simulink model "Tractor_HIT_Discrete"  (R2024a)
settings: Solver=ode1  StartTime=0.0  StopTime=60  FixedStep=0.001  RelTol=1e-3
values from neighbouring files (symbols this model uses):
  ANRtarget = 1.05    [Engine1204.sldd]    (also in Engine1204_init_r1.m; Engine2004.sldd; Engine2004_init.m; Engine3204.sldd)
  BackPrs = 3.0 4.2 5.5 7.0 8.5 10.0 11.5 12.5    [Engine1204.sldd]    (also in Engine1204_init_r1.m = [3.0, 4.2, 5.5, 7.0, 8.5, 10.0, 11.5, 12.5]; Engine2004.sldd = 3.0 4.2 5.5 7.0 8.5 10.0 11.5 12.5 13.5 14.5 15.0 15.5 16.0 ; Engine2004_init.m = [3.0,4.2,5.5,7.0,8.5,10.0,11.5,12.5,13.5,14.5,15.0,15.5,16.0; Engine3204.sldd = 3.0 4.5 6.0 7.5 9.0 10.5 12.0 13.0 13.8 14.4 14.8 15.2 15.6 )
  BackPrs_x = 50.0 100.0 150.0 200.0 250.0 300.0 350.0 400.0    [Engine1204.sldd]    (also in Engine1204_init_r1.m = [50:50:400]; Engine2004.sldd = 50.0 100.0 150.0 200.0 250.0 300.0 350.0 400.0 450.0 500.0 5; Engine2004_init.m = [50:50:800]; Engine3204.sldd = 100.0 200.0 300.0 400.0 500.0 600.0 700.0 800.0 900.0 1000.0)
  Bf = 0.38    [Engine1204.sldd]    (also in Engine2004.sldd; Engine3204.sldd)
  Br = 0.47    [Engine1204.sldd]    (also in Engine2004.sldd; Engine3204.sldd)
  BSFC = 320.0 285.0 275.0 280.0 290.0 300.0 310.0 260.0 225.0 215.0 220.0 228.0 240.0 250.0 235.0 208.0 202.0 205.0 212.0 222.0 232.0 230.0 205.0 200.0 204.0 210.0 220.0 230.0 232.0 207.0 203.0 206.0 213.0 224.0 235.0    [Engine1204.sldd]    (also in Engine1204_init_r1.m = [320,285,275,280,290,300,310; Engine2004.sldd = 315.0 280.0 270.0 275.0 285.0 295.0 305.0 255.0 220.0 210.0 ; Engine2004_init.m = [315,280,270,275,285,295,305; Engine3204.sldd = 310.0 275.0 265.0 270.0 280.0 290.0 300.0 250.0 215.0 205.0 )
  BSFC_x = 700.0 1200.0 1400.0 1600.0 1800.0 2000.0 2200.0    [Engine1204.sldd]    (also in Engine1204_init_r1.m = [700,1200,1400,1600,1800,2000,2200]; Engine2004.sldd = 800.0 1200.0 1400.0 1600.0 1800.0 2000.0 2200.0; Engine2004_init.m = [800,1200,1400,1600,1800,2000,2200]; Engine3204.sldd = 800.0 1000.0 1200.0 1400.0 1600.0 1800.0 2100.0)
  BSFC_y = 12.0 24.0 36.0 48.0 54.0    [Engine1204.sldd]    (also in Engine1204_init_r1.m = [12,24,36,48,54]; Engine2004.sldd = 20.0 40.0 60.0 80.0 100.0; Engine2004_init.m = [20,40,60,80,100]; Engine3204.sldd = 30.0 60.0 90.0 120.0 150.0)
  CO = 2.4 1.7 1.5 1.6 1.8 2.1 2.7 1.1 0.72 0.65 0.68 0.78 0.92 1.3 0.7 0.55 0.5 0.53 0.6 0.72 0.95 1.2 0.9 0.85 0.88 0.96 1.1 1.45 3.2 2.3 2.1 2.25 2.5 2.85 3.8    [Engine1204.sldd]    (also in Engine1204_init_r1.m = [; Engine2004.sldd = 2.3 1.63 1.44 1.54 1.73 2.02 2.56 1.05 0.68 0.61 0.64 0.74 0; Engine2004_init.m = [; Engine3204.sldd = 2.2 1.56 1.38 1.48 1.66 1.94 2.46 1.0 0.65 0.58 0.61 0.7 0.8)
  CO_x = 700.0 1200.0 1400.0 1600.0 1800.0 2000.0 2200.0    [Engine1204.sldd]    (also in Engine1204_init_r1.m = [700,1200,1400,1600,1800,2000,2200]; Engine2004.sldd = 800.0 1200.0 1400.0 1600.0 1800.0 2000.0 2200.0; Engine2004_init.m = [800,1200,1400,1600,1800,2000,2200]; Engine3204.sldd = 800.0 1000.0 1200.0 1400.0 1600.0 1800.0 2100.0)
  CO_y = 12.0 24.0 36.0 48.0 54.0    [Engine1204.sldd]    (also in Engine1204_init_r1.m = [12,24,36,48,54]; Engine2004.sldd = 20.0 40.0 60.0 80.0 100.0; Engine2004_init.m = [20,40,60,80,100]; Engine3204.sldd = 30.0 60.0 90.0 120.0 150.0)
  Df = 1.4    [Engine1204.sldd]    (also in Engine2004.sldd; Engine3204.sldd)
  dfmax = 0.1    [Engine1204.sldd]    (also in Engine2004.sldd; Engine3204.sldd)
  dfmin = 0.035    [Engine1204.sldd]    (also in Engine2004.sldd; Engine3204.sldd)
  DOCdPrs = 0.2 0.5 0.8 1.1 1.2    [Engine1204.sldd]    (also in Engine1204_init_r1.m = [0.2  0.5  0.8  1.1  1.2]; Engine2004.sldd = 0.25 0.55 0.85 1.15 1.3; Engine2004_init.m = [0.25,0.55,0.85,1.15,1.30]; Engine3204.sldd = 0.25 0.55 0.85 1.15 1.3 1.45)
  DOCdPrs_x = 50.0 150.0 250.0 350.0 400.0    [Engine1204.sldd]    (also in Engine1204_init_r1.m = [50  150  250  350  400]; Engine2004.sldd = 100.0 250.0 400.0 600.0 800.0; Engine2004_init.m = [100 250 400 600 800]; Engine3204.sldd = 100.0 250.0 400.0 600.0 800.0 1200.0)
  DPFdPrs = 0.3 0.5 0.7 0.9 0.6 1.0 1.4 1.8 0.9 1.5 2.1 2.6 1.2 2.0 2.7 2.8    [Engine1204.sldd]    (also in Engine1204_init_r1.m = [0.3  0.5  0.7  0.9; Engine2004.sldd = 0.35 0.6 0.85 1.1 0.7 1.15 1.6 2.0 1.05 1.7 2.3 2.5 1.4 2.2 ; Engine2004_init.m = [0.35,0.60,0.85,1.10; Engine3204.sldd = 0.35 0.7 1.05 1.4 1.7 2.0 2.2 2.4 2.55 2.65 2.7 2.75 0.6 1.1)
  DPFdPrs_x = 100.0 200.0 300.0 400.0    [Engine1204.sldd]    (also in Engine1204_init_r1.m = [100: 100 : 400]; Engine2004.sldd = 100.0 300.0 500.0 700.0; Engine2004_init.m = [100:200:700]; Engine3204.sldd = 100.0 200.0 300.0 400.0 500.0 600.0 700.0 800.0 900.0 1000.0)
  DPFdPrs_y = 0.0 6.0 12.0 20.0    [Engine1204.sldd]    (also in Engine1204_init_r1.m = [0 6 12 20 ]; Engine2004.sldd = 0.0 8.0 16.0 24.0; Engine2004_init.m = [0 8 16 24]; Engine3204.sldd = 0.0 10.0 20.0 30.0)
  DPFSootBurn = 0.0 0.0 0.0 0.0 0.0 0.2 0.4 0.6 0.8 1.0 1.2 2.4 3.6 4.8 6.0 6.0 12.0 18.0 24.0 30.0 12.0 24.0 36.0 48.0 60.0 20.0 40.0 60.0 80.0 100.0 22.0 44.0 66.0 88.0 110.0    [Engine1204.sldd]    (also in Engine1204_init_r1.m = [0,0,0,0,0; Engine2004.sldd = 0.0 0.0 0.0 0.0 0.0 0.5 1.0 1.5 2.0 2.5 3.0 6.0 9.0 12.0 15.; Engine2004_init.m = [0,0,0,0,0; Engine3204.sldd = 0.0 0.0 0.0 0.0 0.0 0.5 1.0 1.5 2.0 2.5 3.0 6.0 9.0 12.0 15.)
  DPFSootBurn_x = 100.0 200.0 300.0 400.0 500.0    [Engine1204.sldd]    (also in Engine1204_init_r1.m = [100,200,300,400,500]; Engine2004.sldd = 200.0 300.0 400.0 500.0 650.0; Engine2004_init.m = [200,300,400,500,650]; Engine3204.sldd = 200.0 300.0 400.0 500.0 650.0)
  DPFSootBurn_y = 400.0 450.0 500.0 550.0 600.0 650.0 680.0    [Engine1204.sldd]    (also in Engine1204_init_r1.m = [400,450,500,550,600,650,680]; Engine2004.sldd; Engine2004_init.m = [400,450,500,550,600,650,680]; Engine3204.sldd)
  Dr = 1.8    [Engine1204.sldd]    (also in Engine2004.sldd; Engine3204.sldd)
  drmax = 0.12    [Engine1204.sldd]    (also in Engine2004.sldd; Engine3204.sldd)
  drmin = 0.04    [Engine1204.sldd]    (also in Engine2004.sldd; Engine3204.sldd)
  EGRKi = 0.03    [Engine1204.sldd]    (also in Engine1204_init_r1.m; Engine2004.sldd; Engine2004_init.m; Engine3204.sldd)
  EGRKp = 3.5999999999999996    [Engine1204.sldd]    (also in Engine1204_init_r1.m = 3.6; Engine2004.sldd; Engine2004_init.m = 3.6; Engine3204.sldd)
  EGRMax = 1.0    [Engine1204.sldd]    (also in Engine1204_init_r1.m = 1; Engine2004.sldd; Engine2004_init.m = 1; Engine3204.sldd)
  EGRMin = 0.0    [Engine1204.sldd]    (also in Engine1204_init_r1.m = 0; Engine2004.sldd; Engine2004_init.m = 0; Engine3204.sldd)
  EGRRatio = 0.0 0.0 0.0 0.0 0.0 0.0 0.0 0.0 0.04 0.03 0.03 0.02 0.02 0.01 0.0 0.08 0.07 0.06 0.05 0.04 0.03 0.0 0.13 0.12 0.11 0.1 0.09 0.08 0.0 0.18 0.17 0.16 0.15 0.14 0.13 0.0 0.22 0.21 0.2 0.19 0.18 0.17    [Engine1204.sldd]    (also in Engine1204_init_r1.m = [; Engine2004.sldd; Engine2004_init.m = [; Engine3204.sldd)
  EGRRatio_x = 700.0 1200.0 1400.0 1600.0 1800.0 2000.0 2200.0    [Engine1204.sldd]    (also in Engine1204_init_r1.m = [700,1200,1400,1600,1800,2000,2200]; Engine2004.sldd = 800.0 1200.0 1400.0 1600.0 1800.0 2000.0 2200.0; Engine2004_init.m = [800,1200,1400,1600,1800,2000,2200]; Engine3204.sldd = 800.0 1000.0 1200.0 1400.0 1600.0 1800.0 2100.0)
  EGRRatio_y = 0.0 20.0 40.0 60.0 80.0 100.0    [Engine1204.sldd]    (also in Engine1204_init_r1.m = [0,20,40,60,80,100]; Engine2004.sldd; Engine2004_init.m = [0,20,40,60,80,100]; Engine3204.sldd)
  EGRTgt = 0.25 0.22 0.2 0.18 0.16 0.12 0.1 0.2 0.18 0.15 0.14 0.12 0.1 0.08 0.12 0.13 0.1 0.09 0.08 0.06 0.04 0.08 0.09 0.07 0.06 0.05 0.03 0.02 0.05 0.06 0.04 0.03 0.02 0.01 0.0    [Engine1204.sldd]    (also in Engine1204_init_r1.m = [0.25,0.22,0.20,0.18,0.16,0.12,0.10; Engine2004.sldd = 0.24 0.21 0.19 0.17 0.15 0.11 0.09 0.19 0.17 0.14 0.13 0.11 ; Engine2004_init.m = [0.24,0.21,0.19,0.17,0.15,0.11,0.09; Engine3204.sldd = 0.23 0.2 0.18 0.16 0.14 0.1 0.08 0.18 0.16 0.13 0.12 0.1 0.0)
  EGRTgt_x = 700.0 1200.0 1400.0 1600.0 1800.0 2000.0 2200.0    [Engine1204.sldd]    (also in Engine1204_init_r1.m = [700,1200,1400,1600,1800,2000,2200]; Engine2004.sldd = 800.0 1200.0 1400.0 1600.0 1800.0 2000.0 2200.0; Engine2004_init.m = [800,1200,1400,1600,1800,2000,2200]; Engine3204.sldd = 800.0 1000.0 1200.0 1400.0 1600.0 1800.0 2100.0)
  EGRTgt_y = 12.0 24.0 36.0 48.0 54.0    [Engine1204.sldd]    (also in Engine1204_init_r1.m = [12,24,36,48,54]; Engine2004.sldd = 20.0 40.0 60.0 80.0 100.0; Engine2004_init.m = [20,40,60,80,100]; Engine3204.sldd = 30.0 60.0 90.0 120.0 150.0)
  EGT = 197.0 257.0 287.0 297.0 287.0 267.0 247.0 267.0 357.0 397.0 407.0 392.0 367.0 347.0 337.0 437.0 472.0 482.0 462.0 437.0 407.0 367.0 477.0 502.0 512.0 492.0 467.0 437.0 377.0 487.0 510.0 520.0 500.0 477.0 447.0    [Engine1204.sldd]    (also in Engine1204_init_r1.m = [470,530,560,570,560,540,520; Engine2004.sldd = 187.0 247.0 277.0 287.0 277.0 257.0 237.0 257.0 347.0 387.0 ; Engine2004_init.m = [460,520,550,560,550,530,510; Engine3204.sldd = 307.0 327.0 338.0 327.0 307.0 277.0 237.0 322.0 337.0 332.0 )
  EGT_x = 700.0 1200.0 1400.0 1600.0 1800.0 2000.0 2200.0    [Engine1204.sldd]    (also in Engine1204_init_r1.m = [700,1200,1400,1600,1800,2000,2200]; Engine2004.sldd = 800.0 1200.0 1400.0 1600.0 1800.0 2000.0 2200.0; Engine2004_init.m = [800,1200,1400,1600,1800,2000,2200]; Engine3204.sldd = 800.0 1000.0 1200.0 1400.0 1600.0 1800.0 2100.0)
  EGT_y = 12.0 24.0 36.0 48.0 54.0    [Engine1204.sldd]    (also in Engine1204_init_r1.m = [12,24,36,48,54]; Engine2004.sldd = 20.0 40.0 60.0 80.0 100.0; Engine2004_init.m = [20,40,60,80,100]; Engine3204.sldd = 30.0 60.0 90.0 120.0 150.0)
  EngCsup = 0.35594 0.35501499999999997 0.353535 0.35242500000000004 0.351685 0.35150000000000003 0.35187 0.352795 0.35446 0.356865    [Engine1204.sldd]    (also in Engine2004.sldd; Engine3204.sldd)
  EngineSpdTgt = 700.0 850.0 1000.0 1150.0 1300.0 1450.0 1600.0 1750.0 1900.0 2050.0 2200.0    [Engine1204.sldd]    (also in Engine1204_init_r1.m = [700:150:2200]; Engine2004.sldd; Engine2004_init.m = [700:150:2200]; Engine3204.sldd = 800.0 930.0 1060.0 1190.0 1320.0 1450.0 1580.0 1710.0 1840.0)
  EngineSpdTgt_x = 0.0 10.0 20.0 30.0 40.0 50.0 60.0 70.0 80.0 90.0 100.0    [Engine1204.sldd]    (also in Engine1204_init_r1.m = [0:10:100]; Engine2004.sldd; Engine2004_init.m = [0:10:100]; Engine3204.sldd)
  EngineTrq = 70.0 110.0 130.0 125.0 115.0 100.0 85.0 180.0 280.0 320.0 310.0 285.0 250.0 220.0 260.0 370.0 410.0 395.0 365.0 320.0 280.0 300.0 420.0 450.0 435.0 400.0 350.0 300.0 310.0 435.0 460.0 445.0 410.0 355.0 305.0    [Engine1204.sldd]    (also in Engine1204_init_r1.m = [70,110,130,125,115,100,85; Engine2004.sldd = 130.0 200.0 240.0 230.0 210.0 180.0 150.0 320.0 480.0 550.0 ; Engine2004_init.m = [130,200,240,230,210,180,150; Engine3204.sldd = 210.0 320.0 380.0 360.0 330.0 290.0 240.0 510.0 760.0 870.0 )
  EngineTrq_x = 700.0 1200.0 1400.0 1600.0 1800.0 2000.0 2200.0    [Engine1204.sldd]    (also in Engine1204_init_r1.m = [700,1200,1400,1600,1800,2000,2200]; Engine2004.sldd = 800.0 1200.0 1400.0 1600.0 1800.0 2000.0 2200.0; Engine2004_init.m = [800,1200,1400,1600,1800,2000,2200]; Engine3204.sldd = 800.0 1000.0 1200.0 1400.0 1600.0 1800.0 2100.0)
  EngineTrq_y = 12.0 24.0 36.0 48.0 54.0    [Engine1204.sldd]    (also in Engine1204_init_r1.m = [12,24,36,48,54]; Engine2004.sldd = 20.0 40.0 60.0 80.0 100.0; Engine2004_init.m = [20,40,60,80,100]; Engine3204.sldd = 30.0 60.0 90.0 120.0 150.0)
  EngSpd = 800.0 1000.0 1200.0 1400.0 1600.0 1800.0 2000.0 2200.0 2400.0 2600.0    [Engine1204.sldd]    (also in Engine2004.sldd; Engine3204.sldd)
  EngTrq = 667.0 700.0 768.0 830.0 885.0 860.0 789.0 690.0 542.0 352.0    [Engine1204.sldd]    (also in Engine2004.sldd; Engine3204.sldd)
  etaCO = 0.0 0.0 0.0 0.0 0.6 0.45 0.3 0.15 0.92 0.85 0.75 0.6 0.98 0.95 0.9 0.82 0.99 0.97 0.94 0.88    [Engine1204.sldd]    (also in Engine1204_init_r1.m = [0.00	0.00	0.00	0.00; Engine2004.sldd; Engine2004_init.m = [0.00	0.00	0.00	0.00; Engine3204.sldd)
  etaCO_x = 10000.0 25000.0 40000.0 60000.0    [Engine1204.sldd]    (also in Engine1204_init_r1.m = [10000  25000  40000  60000]; Engine2004.sldd; Engine2004_init.m = [10000 25000 40000 60000]; Engine3204.sldd)
  etaCO_y = 120.0 200.0 280.0 360.0 450.0    [Engine1204.sldd]    (also in Engine1204_init_r1.m = [120, 200, 280, 360, 450]; Engine2004.sldd; Engine2004_init.m = [120,200,280,360,450]; Engine3204.sldd)
  etaHC = 0.0 0.0 0.0 0.0 0.5 0.35 0.2 0.1 0.88 0.8 0.68 0.5 0.96 0.92 0.86 0.75 0.98 0.95 0.91 0.83    [Engine1204.sldd]    (also in Engine1204_init_r1.m = [0.00	0.00	0.00	0.00; Engine2004.sldd; Engine2004_init.m = [0.00	0.00	0.00	0.00; Engine3204.sldd)
  etaHC_x = 10000.0 25000.0 40000.0 60000.0    [Engine1204.sldd]    (also in Engine1204_init_r1.m = [10000  25000  40000  60000]; Engine2004.sldd; Engine2004_init.m = [10000 25000 40000 60000]; Engine3204.sldd)
  etaHC_y = 120.0 200.0 280.0 360.0 450.0    [Engine1204.sldd]    (also in Engine1204_init_r1.m = [120, 200, 280, 360, 450]; Engine2004.sldd; Engine2004_init.m = [120,200,280,360,450]; Engine3204.sldd)
  etaNO2 = 0.0 0.0 0.0 0.0 0.2 0.15 0.1 0.05 0.4 0.33 0.25 0.18 0.55 0.48 0.4 0.3 0.6 0.53 0.45 0.35    [Engine1204.sldd]    (also in Engine1204_init_r1.m = [0.00	0.00	0.00	0.00; Engine2004.sldd; Engine2004_init.m = [0.00	0.00	0.00	0.00; Engine3204.sldd)
  etaNO2_x = 10000.0 25000.0 40000.0 60000.0    [Engine1204.sldd]    (also in Engine1204_init_r1.m = [10000  25000  40000  60000]; Engine2004.sldd; Engine2004_init.m = [10000 25000 40000 60000]; Engine3204.sldd)
  etaNO2_y = 120.0 200.0 280.0 360.0 450.0    [Engine1204.sldd]    (also in Engine1204_init_r1.m = [120, 200, 280, 360, 450]; Engine2004.sldd; Engine2004_init.m = [120,200,280,360,450]; Engine3204.sldd)
  etaPM = 0.995 0.992 0.988 0.98 0.996 0.994 0.99 0.985 0.997 0.995 0.992 0.988    [Engine1204.sldd]    (also in Engine1204_init_r1.m = [0.995  0.992  0.988  0.980; Engine2004.sldd; Engine2004_init.m = [0.995  0.992  0.988  0.980; Engine3204.sldd)
  etaPM_x = 10000.0 25000.0 40000.0 60000.0    [Engine1204.sldd]    (also in Engine1204_init_r1.m = [10000  25000  40000  60000]; Engine2004.sldd; Engine2004_init.m = [10000 25000 40000 60000]; Engine3204.sldd)
  etaPM_y = 150.0 300.0 450.0    [Engine1204.sldd]    (also in Engine1204_init_r1.m = [150, 300, 450]; Engine2004.sldd; Engine2004_init.m = [150,300,450]; Engine3204.sldd)
  FuelCyleMax = 40.0 45.0 50.0 52.0 54.0 50.0 60.0 65.0 66.0 68.0 52.0 64.0 66.0 67.0 68.0 50.0 62.0 64.0 65.0 66.0 48.0 58.0 60.0 61.0 62.0 42.0 50.0 52.0 53.0 54.0 38.0 44.0 46.0 47.0 48.0    [Engine1204.sldd]    (also in Engine1204_init_r1.m = [40,45,50,52,54; Engine2004.sldd = 65.0 75.0 82.0 88.0 92.0 75.0 88.0 94.0 98.0 102.0 78.0 92.0; Engine2004_init.m = [65,75,82,88,92; Engine3204.sldd = 95.0 110.0 125.0 140.0 155.0 110.0 130.0 145.0 160.0 175.0 1)
  FuelCyleMax_x = 80.0 140.0 200.0 260.0 320.0    [Engine1204.sldd]    (also in Engine1204_init_r1.m = [80,140,200,260,320]; Engine2004.sldd = 150.0 300.0 450.0 600.0 750.0; Engine2004_init.m = [150,300,450,600,750]; Engine3204.sldd = 250.0 500.0 750.0 1000.0 1300.0)
  FuelCyleMax_y = 700.0 1200.0 1400.0 1600.0 1800.0 2000.0 2200.0    [Engine1204.sldd]    (also in Engine1204_init_r1.m = [700,1200,1400,1600,1800,2000,2200]; Engine2004.sldd = 800.0 1200.0 1400.0 1600.0 1800.0 2000.0 2200.0; Engine2004_init.m = [800,1200,1400,1600,1800,2000,2200]; Engine3204.sldd = 800.0 1000.0 1200.0 1400.0 1600.0 1800.0 2100.0)
  FuelCyleMaxSw = 0.0    [Engine1204.sldd]    (also in Engine1204_init_r1.m = 0; Engine2004.sldd; Engine2004_init.m = 0; Engine3204.sldd)
  FuelCyleMin = 10.0    [Engine1204.sldd]    (also in Engine1204_init_r1.m = 10; Engine2004.sldd = 12.0; Engine2004_init.m = 12; Engine3204.sldd = 15.0)
  FuelKd = 0.0    [Engine1204.sldd]    (also in Engine1204_init_r1.m = 0; Engine2004.sldd; Engine2004_init.m = 0; Engine3204.sldd)
  FuelKi = 0.0162    [Engine1204.sldd]    (also in Engine1204_init_r1.m; Engine2004.sldd = 0.0198; Engine2004_init.m = 0.0198; Engine3204.sldd = 0.025199999999999997)
  FuelKp = 0.054    [Engine1204.sldd]    (also in Engine1204_init_r1.m; Engine2004.sldd = 0.066; Engine2004_init.m = 0.066; Engine3204.sldd = 0.083999999999999991)
  g = 9.81    [Engine1204.sldd]    (also in Engine2004.sldd; Engine3204.sldd)
  GearA = -2.9 0.0 6.0 2.5 1.0    [Engine1204.sldd]    (also in Engine2004.sldd; Engine3204.sldd)
  GearAC = -1.0 0.0 1.0 2.0 3.0    [Engine1204.sldd]    (also in Engine2004.sldd; Engine3204.sldd)
  GearFront = 17.574    [Engine1204.sldd]    (also in Engine2004.sldd; Engine3204.sldd)
  GearM = 2.33 1.75 1.4 1.0    [Engine1204.sldd]    (also in Engine2004.sldd; Engine3204.sldd)
  GearMC = 1.0 2.0 3.0 4.0    [Engine1204.sldd]    (also in Engine2004.sldd; Engine3204.sldd)
  GearRef = 14.6    [Engine1204.sldd]    (also in Engine2004.sldd; Engine3204.sldd)
  HC = 0.85 0.6 0.52 0.55 0.62 0.7 0.9 0.4 0.22 0.2 0.21 0.26 0.32 0.48 0.25 0.18 0.17 0.18 0.21 0.26 0.36 0.32 0.24 0.23 0.25 0.28 0.33 0.42 0.55 0.42 0.4 0.43 0.48 0.54 0.68    [Engine1204.sldd]    (also in Engine1204_init_r1.m = [; Engine2004.sldd = 0.82 0.58 0.5 0.53 0.6 0.68 0.87 0.38 0.21 0.19 0.2 0.24 0.3; Engine2004_init.m = [; Engine3204.sldd = 0.8 0.56 0.48 0.51 0.58 0.66 0.84 0.37 0.2 0.18 0.19 0.23 0.)
  HC_x = 700.0 1200.0 1400.0 1600.0 1800.0 2000.0 2200.0    [Engine1204.sldd]    (also in Engine1204_init_r1.m = [700,1200,1400,1600,1800,2000,2200]; Engine2004.sldd = 800.0 1200.0 1400.0 1600.0 1800.0 2000.0 2200.0; Engine2004_init.m = [800,1200,1400,1600,1800,2000,2200]; Engine3204.sldd = 800.0 1000.0 1200.0 1400.0 1600.0 1800.0 2100.0)
  HC_y = 12.0 24.0 36.0 48.0 54.0    [Engine1204.sldd]    (also in Engine1204_init_r1.m = [12,24,36,48,54]; Engine2004.sldd = 20.0 40.0 60.0 80.0 100.0; Engine2004_init.m = [20,40,60,80,100]; Engine3204.sldd = 30.0 60.0 90.0 120.0 150.0)
  hf = 0.35    [Engine1204.sldd]    (also in Engine2004.sldd; Engine3204.sldd)
  hr = 0.4    [Engine1204.sldd]    (also in Engine2004.sldd; Engine3204.sldd)
  IdleEngSpd = 700.0    [Engine1204.sldd]    (also in Engine2004.sldd; Engine3204.sldd)
  IdleThrottle = 0.3    [Engine1204.sldd]    (also in Engine2004.sldd; Engine3204.sldd)
  Inertia = 0.9    [Engine1204.sldd]    (also in Engine1204_init_r1.m; Engine2004.sldd = 1.4; Engine2004_init.m = 1.4; Engine3204.sldd = 2.0)
  Intake = 80.0 140.0 160.0 180.0 190.0 195.0 200.0 130.0 210.0 240.0 260.0 270.0 275.0 280.0 170.0 270.0 310.0 330.0 340.0 345.0 350.0 190.0 320.0 360.0 380.0 390.0 395.0 400.0 200.0 340.0 380.0 400.0 410.0 415.0 420.0    [Engine1204.sldd]    (also in Engine1204_init_r1.m = [80,140,160,180,190,195,200; Engine2004.sldd = 160.0 240.0 280.0 310.0 330.0 340.0 350.0 250.0 380.0 440.0 ; Engine2004_init.m = [160,240,280,310,330,340,350; Engine3204.sldd = 280.0 420.0 490.0 540.0 570.0 585.0 600.0 430.0 660.0 760.0 )
  Intake_x = 700.0 1200.0 1400.0 1600.0 1800.0 2000.0 2200.0    [Engine1204.sldd]    (also in Engine1204_init_r1.m = [700,1200,1400,1600,1800,2000,2200]; Engine2004.sldd = 800.0 1200.0 1400.0 1600.0 1800.0 2000.0 2200.0; Engine2004_init.m = [800,1200,1400,1600,1800,2000,2200]; Engine3204.sldd = 800.0 1000.0 1200.0 1400.0 1600.0 1800.0 2100.0)
  Intake_y = 12.0 24.0 36.0 48.0 54.0    [Engine1204.sldd]    (also in Engine1204_init_r1.m = [12,24,36,48,54]; Engine2004.sldd = 20.0 40.0 60.0 80.0 100.0; Engine2004_init.m = [20,40,60,80,100]; Engine3204.sldd = 30.0 60.0 90.0 120.0 150.0)
  IntakePrs = 1.0 1.1 1.22 1.35 1.48 1.6 1.7 1.0 1.12 1.24 1.37 1.5 1.62 1.72 1.0 1.13 1.25 1.38 1.51 1.63 1.73 1.0 1.14 1.26 1.39 1.52 1.64 1.74 1.0 1.15 1.27 1.4 1.53 1.65 1.75 1.0 1.16 1.28 1.41 1.54 1.66 1.76    [Engine1204.sldd]    (also in Engine1204_init_r1.m = [; Engine2004.sldd = 1.0 1.11 1.23 1.36 1.49 1.61 1.71 1.0 1.13 1.25 1.38 1.51 1.; Engine2004_init.m = [; Engine3204.sldd = 1.0 1.12 1.24 1.37 1.5 1.62 1.72 1.0 1.14 1.26 1.39 1.52 1.6)
  IntakePrs_x = 700.0 1200.0 1400.0 1600.0 1800.0 2000.0 2200.0    [Engine1204.sldd]    (also in Engine1204_init_r1.m = [700,1200,1400,1600,1800,2000,2200]; Engine2004.sldd = 800.0 1200.0 1400.0 1600.0 1800.0 2000.0 2200.0; Engine2004_init.m = [800,1200,1400,1600,1800,2000,2200]; Engine3204.sldd = 800.0 1000.0 1200.0 1400.0 1600.0 1800.0 2100.0)
  IntakePrs_y = 0.0 20.0 40.0 60.0 80.0 100.0    [Engine1204.sldd]    (also in Engine1204_init_r1.m = [0,20,40,60,80,100]; Engine2004.sldd; Engine2004_init.m = [0,20,40,60,80,100]; Engine3204.sldd)
  IntakePrsInit = 1.35    [Engine1204.sldd]    (also in Engine1204_init_r1.m; Engine2004.sldd; Engine2004_init.m; Engine3204.sldd)
  IntakeSw = 0    [Engine1204.sldd]    (also in Engine1204_init_r1.m = false; Engine2004.sldd; Engine2004_init.m = false; Engine3204.sldd)
  IntakeTC = 0.1    [Engine1204.sldd]    (also in Engine1204_init_r1.m; Engine2004.sldd; Engine2004_init.m; Engine3204.sldd)
  IntakeTemp = 25.0 28.0 30.0 32.0 34.0 36.0 38.0 25.0 38.0 40.0 42.0 44.0 46.0 48.0 25.0 48.0 50.0 52.0 54.0 56.0 58.0 25.0 58.0 60.0 62.0 64.0 66.0 68.0 25.0 66.0 68.0 70.0 72.0 74.0 76.0 25.0 72.0 74.0 76.0 78.0 80.0 82.0    [Engine1204.sldd]    (also in Engine1204_init_r1.m = [; Engine2004.sldd = 25.0 29.0 31.0 33.0 35.0 37.0 39.0 25.0 39.0 41.0 43.0 45.0 ; Engine2004_init.m = [; Engine3204.sldd = 25.0 30.0 32.0 34.0 36.0 38.0 40.0 25.0 40.0 42.0 44.0 46.0 )
  IntakeTemp_x = 700.0 1200.0 1400.0 1600.0 1800.0 2000.0 2200.0    [Engine1204.sldd]    (also in Engine1204_init_r1.m = [700,1200,1400,1600,1800,2000,2200]; Engine2004.sldd = 800.0 1200.0 1400.0 1600.0 1800.0 2000.0 2200.0; Engine2004_init.m = [800,1200,1400,1600,1800,2000,2200]; Engine3204.sldd = 800.0 1000.0 1200.0 1400.0 1600.0 1800.0 2100.0)
  IntakeTemp_y = 0.0 20.0 40.0 60.0 80.0 100.0    [Engine1204.sldd]    (also in Engine1204_init_r1.m = [0,20,40,60,80,100]; Engine2004.sldd; Engine2004_init.m = [0,20,40,60,80,100]; Engine3204.sldd)
  IntakeTempInit = 45.0    [Engine1204.sldd]    (also in Engine1204_init_r1.m = 45; Engine2004.sldd; Engine2004_init.m = 45; Engine3204.sldd)
  Jf = 180.0    [Engine1204.sldd]    (also in Engine2004.sldd; Engine3204.sldd)
  Jr = 450.0    [Engine1204.sldd]    (also in Engine2004.sldd; Engine3204.sldd)
  L = 2.75    [Engine1204.sldd]    (also in Engine2004.sldd; Engine3204.sldd)
  LiftTorque = 5000.0    [Engine1204.sldd]    (also in Engine2004.sldd; Engine3204.sldd)
  LoadTrqManu = 200.0    [Engine1204.sldd]    (also in Engine1204_init_r1.m = 200; Engine2004.sldd = 400.0; Engine2004_init.m = 400; Engine3204.sldd = 800.0)
  LoadTrqSW = 1    [Engine1204.sldd]    (also in Engine1204_init_r1.m = true; Engine2004.sldd; Engine2004_init.m = true; Engine3204.sldd = 0)
  M_I = 2500.0    [Engine1204.sldd]    (also in Engine2004.sldd; Engine3204.sldd)
  M_T = 6500.0    [Engine1204.sldd]    (also in Engine2004.sldd; Engine3204.sldd)
  MaxEngSpd = 2600.0    [Engine1204.sldd]    (also in Engine2004.sldd; Engine3204.sldd)
  NH3StoreMax = 0.0 1.2 2.0 2.4 2.2 1.7 1.1    [Engine1204.sldd]    (also in Engine1204_init_r1.m = [0  1.2  2.0  2.4  2.2  1.7  1.1]; Engine2004.sldd = 0.0 1.7 2.9 3.5 3.2 2.5 1.6; Engine2004_init.m = [0, 1.7, 2.9, 3.5, 3.2, 2.5, 1.6]; Engine3204.sldd = 0.0 2.2 3.8 4.5 4.2 3.3 2.1)
  NH3StoreMax_x = 180.0 220.0 260.0 300.0 340.0 380.0 420.0    [Engine1204.sldd]    (also in Engine1204_init_r1.m = [180  220  260  300  340  380  420]; Engine2004.sldd; Engine2004_init.m = [180 220 260 300 340 380 420]; Engine3204.sldd)
  NOx = 6.2 7.0 7.4 7.2 6.8 6.4 6.0 7.5 8.4 8.8 8.6 8.2 7.7 7.2 8.2 9.1 9.5 9.3 8.9 8.4 7.9 7.6 8.5 8.8 8.6 8.2 7.7 7.2 7.0 7.8 8.1 7.9 7.5 7.0 6.5    [Engine1204.sldd]    (also in Engine1204_init_r1.m = [6.2,7.0,7.4,7.2,6.8,6.4,6.0; Engine2004.sldd = 6.1 6.9 7.3 7.1 6.7 6.3 5.9 7.4 8.3 8.7 8.5 8.1 7.6 7.1 8.1 ; Engine2004_init.m = [6.1,6.9,7.3,7.1,6.7,6.3,5.9; Engine3204.sldd = 5.9 6.7 7.1 6.9 6.5 6.1 5.7 7.2 8.1 8.5 8.3 7.9 7.4 6.9 7.9 )
  NOx_x = 700.0 1200.0 1400.0 1600.0 1800.0 2000.0 2200.0    [Engine1204.sldd]    (also in Engine1204_init_r1.m = [700,1200,1400,1600,1800,2000,2200]; Engine2004.sldd = 800.0 1200.0 1400.0 1600.0 1800.0 2000.0 2200.0; Engine2004_init.m = [800,1200,1400,1600,1800,2000,2200]; Engine3204.sldd = 800.0 1000.0 1200.0 1400.0 1600.0 1800.0 2100.0)
  NOx_y = 12.0 24.0 36.0 48.0 54.0    [Engine1204.sldd]    (also in Engine1204_init_r1.m = [12,24,36,48,54]; Engine2004.sldd = 20.0 40.0 60.0 80.0 100.0; Engine2004_init.m = [20,40,60,80,100]; Engine3204.sldd = 30.0 60.0 90.0 120.0 150.0)
  NOxFac = 1.0 0.88 0.76 0.64 0.54 0.46 0.4    [Engine1204.sldd]    (also in Engine1204_init_r1.m = [1.00, 0.88, 0.76, 0.64, 0.54, 0.46, 0.40]; Engine2004.sldd; Engine2004_init.m = [1.00,0.88,0.76,0.64,0.54,0.46,0.40]; Engine3204.sldd)
  NOxFac_x = 0.0 0.05 0.1 0.15 0.19999999999999998 0.25 0.3    [Engine1204.sldd]    (also in Engine1204_init_r1.m = [0: 0.05 : 0.3]; Engine2004.sldd; Engine2004_init.m = [0:0.05:0.3]; Engine3204.sldd)
  NumCyl = 6.0    [Engine1204.sldd]    (also in Engine1204_init_r1.m = 6; Engine2004.sldd; Engine2004_init.m = 6; Engine3204.sldd)
  O2 = 16.5 16.0 15.8 15.5 15.2 14.8 14.5 13.0 12.2 11.8 11.5 11.2 10.8 10.5 9.5 8.6 8.0 7.7 7.4 7.0 6.7 7.0 6.2 5.6 5.3 5.0 4.7 4.4 6.0 5.3 4.8 4.5 4.2 4.0 3.8    [Engine1204.sldd]    (also in Engine1204_init_r1.m = [16.5,16.0,15.8,15.5,15.2,14.8,14.5; Engine2004.sldd = 16.3 15.8 15.6 15.3 15.0 14.6 14.3 12.8 12.0 11.6 11.3 11.0 ; Engine2004_init.m = [16.3,15.8,15.6,15.3,15.0,14.6,14.3; Engine3204.sldd = 16.0 15.5 15.3 15.0 14.7 14.3 14.0 12.5 11.7 11.3 11.0 10.7 )
  O2_x = 700.0 1200.0 1400.0 1600.0 1800.0 2000.0 2200.0    [Engine1204.sldd]    (also in Engine1204_init_r1.m = [700,1200,1400,1600,1800,2000,2200]; Engine2004.sldd = 800.0 1200.0 1400.0 1600.0 1800.0 2000.0 2200.0; Engine2004_init.m = [800,1200,1400,1600,1800,2000,2200]; Engine3204.sldd = 800.0 1000.0 1200.0 1400.0 1600.0 1800.0 2100.0)
  O2_y = 12.0 24.0 36.0 48.0 54.0    [Engine1204.sldd]    (also in Engine1204_init_r1.m = [12,24,36,48,54]; Engine2004.sldd = 20.0 40.0 60.0 80.0 100.0; Engine2004_init.m = [20,40,60,80,100]; Engine3204.sldd = 30.0 60.0 90.0 120.0 150.0)
  PM = 0.12 0.1 0.09 0.09 0.1 0.11 0.12 0.22 0.18 0.16 0.17 0.19 0.21 0.24 0.38 0.3 0.26 0.27 0.31 0.35 0.39 0.55 0.44 0.38 0.4 0.45 0.5 0.56 0.65 0.52 0.46 0.48 0.53 0.58 0.66    [Engine1204.sldd]    (also in Engine1204_init_r1.m = [0.12,0.10,0.09,0.09,0.10,0.11,0.12; Engine2004.sldd = 0.11 0.09 0.08 0.08 0.09 0.1 0.11 0.21 0.17 0.15 0.16 0.18 0; Engine2004_init.m = [0.11,0.09,0.08,0.08,0.09,0.10,0.11; Engine3204.sldd = 0.1 0.08 0.07 0.07 0.08 0.09 0.1 0.2 0.16 0.14 0.15 0.17 0.1)
  PM_x = 700.0 1200.0 1400.0 1600.0 1800.0 2000.0 2200.0    [Engine1204.sldd]    (also in Engine1204_init_r1.m = [700,1200,1400,1600,1800,2000,2200]; Engine2004.sldd = 800.0 1200.0 1400.0 1600.0 1800.0 2000.0 2200.0; Engine2004_init.m = [800,1200,1400,1600,1800,2000,2200]; Engine3204.sldd = 800.0 1000.0 1200.0 1400.0 1600.0 1800.0 2100.0)
  PM_y = 12.0 24.0 36.0 48.0 54.0    [Engine1204.sldd]    (also in Engine1204_init_r1.m = [12,24,36,48,54]; Engine2004.sldd = 20.0 40.0 60.0 80.0 100.0; Engine2004_init.m = [20,40,60,80,100]; Engine3204.sldd = 30.0 60.0 90.0 120.0 150.0)
  radps2rpm = 9.55    [Engine1204.sldd]    (also in Engine1204_init_r1.m; Engine2004.sldd; Engine2004_init.m; Engine3204.sldd)
  RailFuel = 400.0 600.0 700.0 700.0 650.0 600.0 550.0 600.0 800.0 900.0 900.0 850.0 800.0 750.0 700.0 1000.0 1100.0 1150.0 1100.0 1000.0 950.0 750.0 1200.0 1350.0 1350.0 1300.0 1200.0 1150.0 750.0 1300.0 1400.0 1450.0 1400.0 1300.0 1200.0    [Engine1204.sldd]    (also in Engine1204_init_r1.m = [400,600,700,700,650,600,550; Engine2004.sldd = 420.0 620.0 720.0 720.0 680.0 630.0 580.0 630.0 830.0 930.0 ; Engine2004_init.m = [420,620,720,720,680,630,580; Engine3204.sldd = 440.0 640.0 740.0 740.0 700.0 650.0 600.0 650.0 850.0 950.0 )
  RailFuel_x = 700.0 1200.0 1400.0 1600.0 1800.0 2000.0 2200.0    [Engine1204.sldd]    (also in Engine1204_init_r1.m = [700,1200,1400,1600,1800,2000,2200]; Engine2004.sldd = 800.0 1200.0 1400.0 1600.0 1800.0 2000.0 2200.0; Engine2004_init.m = [800,1200,1400,1600,1800,2000,2200]; Engine3204.sldd = 800.0 1000.0 1200.0 1400.0 1600.0 1800.0 2100.0)
  ... (+23 more)
undefined symbols (not defined in the file or in its folder): df, DiscIntNeverNeededParam, dr, MAP_AIR, MAP_EFF, MAP_EoCO, MAP_EoCO2, MAP_EoHC, MAP_EoNOx, MAP_EoPM, MAP_FUEL, MAP_FUELCMD, MAP_POWER, MAP_SPD, MAP_TEMPERATURE, NH3_MAX, R
libraries: simulink x9, slpidlib x5
(part 9 of 10)

== system Tractor_HIT_Discrete/EngineModel/Engine1/ThermalModel/IntakeSystem ==
  note: EGR 率：再循环废气质量流量，占 进气总质量流量（新鲜空气 + EGR 废气） 的百分比。
  note: 50~150 ms
  note: 流量修正系数
  note: 基础进气量
  FuelCycle_mg : Inport
  EGROpeningTgt_pct : Inport  Port=2
  EngineSpd_rpm : Inport  Port=3
  Add : Sum  Inputs=+-
  Constant : Constant
  Constant1 : Constant  Value=IntakeSw
  Constant2 : Constant  Value=IntakeTempInit
  Constant3 : Constant  Value=IntakePrsInit
  EGRRatioMap : Lookup_n-D  BreakpointsForDimension1=EGRRatio_x  BreakpointsForDimension2=EGRRatio_y  Table=EGRRatio  ExtrapMethod=Clip  InternalRulePriority=Speed  RndMeth=Simplest
      settings: InputPortMap=u0,u1
  IntakeMap : Lookup_n-D  BreakpointsForDimension1=Intake_x  BreakpointsForDimension2=Intake_y  Table=Intake  ExtrapMethod=Clip  InternalRulePriority=Speed  RndMeth=Simplest
      settings: InputPortMap=u0,u1
  IntakePrsMap : Lookup_n-D  BreakpointsForDimension1=IntakePrs_x  BreakpointsForDimension2=IntakePrs_y  Table=IntakePrs  ExtrapMethod=Clip  InternalRulePriority=Speed  RndMeth=Simplest
      settings: InputPortMap=u0,u1
  IntakeTempMap : Lookup_n-D  BreakpointsForDimension1=IntakeTemp_x  BreakpointsForDimension2=IntakeTemp_y  Table=IntakeTemp  ExtrapMethod=Clip  InternalRulePriority=Speed  RndMeth=Simplest
      settings: InputPortMap=u0,u1
  Product : Product
  Scope : Scope  NumInputPorts=6
  Switch : Switch  Criteria=u2 > Threshold  SaturateOnIntegerOverflow=off  InputSameDT=off
  Switch1 : Switch  Criteria=u2 > Threshold  SaturateOnIntegerOverflow=off  InputSameDT=off
  Transfer Fcn : TransferFcn  Denominator=[IntakeTC 1]
  bar2kpa : Gain  Gain=100
  IntakeMass_kg/h : Outport
  IntakeTemp_c : Outport  Port=2
  IntakePrs_kpa : Outport  Port=3
  EGRRatio : Outport  Port=4
  wires:
  IntakeMap/1 -> Product/1
  EngineSpd_rpm/1 -> Scope/1, IntakePrsMap/1, IntakeTempMap/1, EGRRatioMap/1, IntakeMap/1
  FuelCycle_mg/1 -> Scope/2, IntakeMap/2
  Transfer Fcn/1 -> Scope/3, IntakeMass_kg/h/1
  EGROpeningTgt_pct/1 -> IntakePrsMap/2, IntakeTempMap/2, EGRRatioMap/2
  EGRRatioMap/1 -> Add/2, Scope/4, EGRRatio/1
  Constant/1 -> Add/1
  Add/1 -> Product/2
  Product/1 -> Transfer Fcn/1
  IntakeTempMap/1 -> Switch/1
  IntakePrsMap/1 -> Switch1/1
  Switch1/1 -> bar2kpa/1
  Switch/1 -> Scope/5, IntakeTemp_c/1
  Constant1/1 -> Switch1/2, Switch/2
  Constant2/1 -> Switch/3
  Constant3/1 -> Switch1/3
  bar2kpa/1 -> IntakePrs_kpa/1, Scope/6

== system Tractor_HIT_Discrete/WorkloadModel/Agricultural Implement/Chisel Plow4/4 ==
  Velocity : Inport
  TIllageCmd : Inport  Port=2
  A : Constant  Value=91
  Add : Sum  Inputs=+++
  B : Constant  Value=5.4
  Bus Selector : BusSelector  OutputSignals=FiCmd,ToolsCmd,WidthCmd,DepthCmd
  C : Constant  Value=0
  Math Function : Math  Operator=square
  Product{,1..4,6} (6 alike) : Product
  Width[m] : Outport
  draft force : Outport  Port=2
  wires:
  B/1 -> Product1/1
  C/1 -> Product2/1
  Velocity/1 -> Product1/2, Math Function/1
  Math Function/1 -> Product2/2
  A/1 -> Add/1
  Product1/1 -> Add/2
  Product2/1 -> Add/3
  Add/1 -> Product/1
  [DepthCmd] -> Product/2
  Product/1 -> Product3/1
  [ToolsCmd] -> Product6/1, Product3/2
  Product3/1 -> Product4/2
  [FiCmd] -> Product4/1
  Product4/1 -> draft force/1
  Product6/1 -> Width[m]/1
  [WidthCmd] -> Product6/2
  Bus Selector/1 -> [FiCmd]  "<FiCmd>"
  TIllageCmd/1 -> Bus Selector/1
  Bus Selector/3 -> [WidthCmd]  "<WidthCmd>"
  Bus Selector/2 -> [ToolsCmd]  "<ToolsCmd>"
  Bus Selector/4 -> [DepthCmd]  "<DepthCmd>"

== system Tractor_HIT_Discrete/WorkloadModel/Agricultural Implement/Cultivator0/draught ==
  Velocity : Inport
  TIllageCmd : Inport  Port=2
  A : Constant  Value=46
  Add : Sum  Inputs=+++
  B : Constant  Value=2.8
  Bus Selector : BusSelector  OutputSignals=FiCmd,ToolsCmd,WidthCmd,DepthCmd
  C : Constant  Value=0
  Math Function : Math  Operator=square
  Product{,1..4,6} (6 alike) : Product
  Width[m] : Outport
  draft force : Outport  Port=2
  wires:
  B/1 -> Product1/1
  C/1 -> Product2/1
  Velocity/1 -> Product1/2, Math Function/1
  Math Function/1 -> Product2/2
  A/1 -> Add/1
  Product1/1 -> Add/2
  Product2/1 -> Add/3
  Add/1 -> Product/1
  [DepthCmd] -> Product/2
  Product/1 -> Product3/1
  [ToolsCmd] -> Product6/1, Product3/2
  Product3/1 -> Product4/2
  [FiCmd] -> Product4/1
  Product6/1 -> Width[m]/1
  [WidthCmd] -> Product6/2
  Product4/1 -> draft force/1
  TIllageCmd/1 -> Bus Selector/1
  Bus Selector/2 -> [ToolsCmd]  "<ToolsCmd>"
  Bus Selector/3 -> [WidthCmd]  "<WidthCmd>"
  Bus Selector/4 -> [DepthCmd]  "<DepthCmd>"
  Bus Selector/1 -> [FiCmd]  "<FiCmd>"

== system Tractor_HIT_Discrete/WorkloadModel/Agricultural Implement/Moldboard Plow1/1 ==
  Velocity : Inport
  TillageCmd : Inport  Port=2
  A : Constant  Value=652
  Add : Sum  Inputs=+++
  B : Constant  Value=0
  Bus Selector : BusSelector  OutputSignals=FiCmd,ToolsCmd,WidthCmd,DepthCmd
  C : Constant  Value=5.1
  Math Function : Math  Operator=square
  Product{,1..4,6} (6 alike) : Product
  Width[m] : Outport
  draft force : Outport  Port=2
  wires:
  B/1 -> Product1/1
  C/1 -> Product2/1
  Velocity/1 -> Product1/2, Math Function/1
  Math Function/1 -> Product2/2
  A/1 -> Add/1
  Product1/1 -> Add/2
  Product2/1 -> Add/3
  Add/1 -> Product/1
  [DepthCmd] -> Product/2
  Product/1 -> Product3/1
  Product3/1 -> Product4/2
  [FiCmd] -> Product4/1
  Product4/1 -> draft force/1
  Product6/1 -> Width[m]/1, Product3/2
  [ToolsCmd] -> Product6/1
  [WidthCmd] -> Product6/2
  Bus Selector/1 -> [FiCmd]  "<FiCmd>"
  Bus Selector/2 -> [ToolsCmd]  "<ToolsCmd>"
  Bus Selector/3 -> [WidthCmd]  "<WidthCmd>"
  Bus Selector/4 -> [DepthCmd]  "<DepthCmd>"
  TillageCmd/1 -> Bus Selector/1

== system Tractor_HIT_Discrete/WorkloadModel/Agricultural Implement/Subsoiler3/3 ==
  Velocity : Inport
  TIllageCmd : Inport  Port=2
  A : Constant  Value=226
  Add : Sum  Inputs=+++
  B : Constant  Value=0
  Bus Selector : BusSelector  OutputSignals=FiCmd,ToolsCmd,WidthCmd,DepthCmd
  C : Constant  Value=1.8
  Math Function : Math  Operator=square
  Product{,1..4,6} (6 alike) : Product
  Width[m] : Outport
  draft force : Outport  Port=2
  wires:
  [FiCmd] -> Product4/1
  Product3/1 -> Product4/2
  [ToolsCmd] -> Product6/1
  Product/1 -> Product3/1
  [DepthCmd] -> Product/2
  Add/1 -> Product/1
  Product2/1 -> Add/3
  Product1/1 -> Add/2
  A/1 -> Add/1
  Math Function/1 -> Product2/2
  Velocity/1 -> Math Function/1, Product1/2
  C/1 -> Product2/1
  B/1 -> Product1/1
  Product4/1 -> draft force/1
  Product6/1 -> Product3/2, Width[m]/1
  [WidthCmd] -> Product6/2
  Bus Selector/1 -> [FiCmd]  "<FiCmd>"
  TIllageCmd/1 -> Bus Selector/1
  Bus Selector/3 -> [WidthCmd]  "<WidthCmd>"
  Bus Selector/2 -> [ToolsCmd]  "<ToolsCmd>"
  Bus Selector/4 -> [DepthCmd]  "<DepthCmd>"

== system Tractor_HIT_Discrete/WorkloadModel/Agricultural Implement/Sweep Plow2/2 ==
  Velocity : Inport
  TIllageCmd : Inport  Port=2
  A : Constant  Value=390
  Add : Sum  Inputs=+++
  B : Constant  Value=19
  Bus Selector : BusSelector  OutputSignals=FiCmd,ToolsCmd,WidthCmd,DepthCmd
  C : Constant  Value=0
  Math Function : Math  Operator=square
  Product{,1..5} (6 alike) : Product
  Width[m] : Outport
  draft force1 : Outport  Port=2
  wires:
  [FiCmd] -> Product4/1
  Product3/1 -> Product4/2
  Product5/1 -> Width[m]/1
  Product/1 -> Product3/1
  [DepthCmd] -> Product/2
  Add/1 -> Product/1
  Product2/1 -> Add/3
  Product1/1 -> Add/2
  A/1 -> Add/1
  Math Function/1 -> Product2/2
  Velocity/1 -> Math Function/1, Product1/2
  C/1 -> Product2/1
  B/1 -> Product1/1
  Product4/1 -> draft force1/1
  [ToolsCmd] -> Product3/2, Product5/1
  [WidthCmd] -> Product5/2
  Bus Selector/1 -> [FiCmd]  "<FiCmd>"
  TIllageCmd/1 -> Bus Selector/1
  Bus Selector/3 -> [WidthCmd]  "<WidthCmd>"
  Bus Selector/2 -> [ToolsCmd]  "<ToolsCmd>"
  Bus Selector/4 -> [DepthCmd]  "<DepthCmd>"

== system Tractor_HIT_Discrete/WorkloadModel/Tires and Ground/Bn_Calc_single/Subsystem2 ==
  CI[Pa] : Inport
  Fzf[N] : Inport  Port=2
  Fzr[N] : Inport  Port=3
  Constant : Constant  Value=Bf
  Constant1 : Constant  Value=Df
  Constant3 : Constant  Value=Br
  Constant4 : Constant  Value=Dr
  Divide : Product  Inputs=*/
  Divide3 : Product  Inputs=*/
  Product : Product  Inputs=3
  Product1 : Product  Inputs=3
  Cn_f : Outport
  Cn_r : Outport  Port=2
  wires:
  Constant3/1 -> Product1/1
  CI[Pa]/1 -> Product1/3, Product/3
  Constant1/1 -> Product/2
  Fzf[N]/1 -> Divide/2
  Fzr[N]/1 -> Divide3/2
  Product1/1 -> Divide3/1
  Constant4/1 -> Product1/2
  Constant/1 -> Product/1
  Product/1 -> Divide/1
  Divide3/1 -> Cn_r/1  "Cn_r"
  Divide/1 -> Cn_f/1  "Cn_f"

== system Tractor_HIT_Discrete/WorkloadModel/Tires and Ground/Bn_Calc_single/旱田 ==
  note: Bn_f_single
  note: Bn_r_single
  Cn_f : Inport
  Cn_r : Inport  Port=2
  Add{1..4} (4 alike) : Sum
  Constant13 : Constant  Value=Df
  Constant15 : Constant  Value=hf
  Constant16 : Constant  Value=Bf
  Constant2 : Constant
  Constant5 : Constant  Value=Dr
  Constant6 : Constant  Value=hr
  Constant7 : Constant  Value=Br
  Constant8 : Constant
  Divide{1..2,4,6} (4 alike) : Product  Inputs=*/
  Divide5 : Product  Inputs=**/
  Divide7 : Product  Inputs=**/
  Gain : Gain  Gain=5
  Gain1 : Gain  Gain=5
  Gain2 : Gain  Gain=3
  Gain3 : Gain  Gain=3
  df : simulink/Sources/Repeating Sequence  rep_seq_t=[0 2]  rep_seq_y=[dfmin dfmax]
  dr : simulink/Sources/Repeating Sequence  rep_seq_t=[0 2]  rep_seq_y=[drmin drmax]
  Bn_f : Outport
  Bn_r : Outport  Port=2
  wires:
  Divide7/1 -> Bn_f/1
  Divide5/1 -> Bn_r/1
  Gain3/1 -> Divide6/1
  Add1/1 -> Divide7/2
  Gain/1 -> Divide1/1
  Cn_f/1 -> Divide7/1
  df/1 -> Gain/1
  Constant13/1 -> Divide6/2
  Constant16/1 -> Gain3/1
  Divide1/1 -> Add1/1
  Divide6/1 -> Add2/2
  Add2/1 -> Divide7/3
  Constant15/1 -> Divide1/2
  Constant2/1 -> Add1/2, Add2/1
  Cn_r/1 -> Divide5/1
  dr/1 -> Gain1/1
  Constant6/1 -> Divide2/2
  Constant7/1 -> Gain2/1
  Add3/1 -> Divide5/2
  Divide4/1 -> Add4/2
  Constant5/1 -> Divide4/2
  Gain2/1 -> Divide4/1
  Gain1/1 -> Divide2/1
  Divide2/1 -> Add3/1
  Add4/1 -> Divide5/3
  Constant8/1 -> Add4/1, Add3/2

== system Tractor_HIT_Discrete/WorkloadModel/Tires and Ground/Bn_Calc_single/水田 ==
  note: Bn_f_single
  note: Bn_r_single
  Cn_f : Inport
  Cn_r : Inport  Port=2
  Add2 : Sum
  Add4 : Sum
  Constant13 : Constant  Value=Df
  Constant15 : Constant  Value=hf
  Constant16 : Constant  Value=Bf
  Constant2 : Constant
  Constant5 : Constant  Value=Dr
  Constant6 : Constant  Value=hr
  Constant7 : Constant  Value=Br
  Constant8 : Constant
  Divide{1..2,4,6} (4 alike) : Product  Inputs=*/
  Divide5 : Product  Inputs=**/
  Divide7 : Product  Inputs=**/
  Gain2 : Gain  Gain=2
  Gain3 : Gain  Gain=2
  Sqrt : Sqrt
  Sqrt1 : Sqrt
  df : simulink/Sources/Repeating Sequence  rep_seq_t=[0 2]  rep_seq_y=[dfmin dfmax]
  dr : simulink/Sources/Repeating Sequence  rep_seq_t=[0 2]  rep_seq_y=[drmin drmax]
  Bn_f : Outport
  Bn_r : Outport  Port=2
  wires:
  Divide7/1 -> Bn_f/1
  Divide5/1 -> Bn_r/1
  Constant16/1 -> Divide6/1
  Sqrt/1 -> Divide7/2
  df/1 -> Divide1/1
  Cn_f/1 -> Divide7/1
  Constant13/1 -> Gain3/1
  Divide1/1 -> Sqrt/1
  Divide6/1 -> Add2/2
  Add2/1 -> Divide7/3
  Constant15/1 -> Divide1/2
  Constant2/1 -> Add2/1
  Cn_r/1 -> Divide5/1
  Constant6/1 -> Divide2/2
  Sqrt1/1 -> Divide5/2
  Divide4/1 -> Add4/2
  Constant5/1 -> Gain2/1
  Constant7/1 -> Divide4/1
  dr/1 -> Divide2/1
  Divide2/1 -> Sqrt1/1
  Add4/1 -> Divide5/3
  Constant8/1 -> Add4/1
  Gain3/1 -> Divide6/2
  Gain2/1 -> Divide4/2

== system Tractor_HIT_Discrete/WorkloadModel/Tires and Ground/CI_Calc/1 ==
  note: %CI=(C1*(DD^C4))/(C2+(MC-C3)^2) Ayers模型
  moisture[%] : Inport
  density[g/cm3] : Inport  Port=2
  Action Port : ActionPort  ActionPortLabel=elseif(u1 == 1)
  Add : Sum
  C1 : Constant  Value=82.39
  C2 : Constant  Value=9.47
  C3 : Constant  Value=4.77
  C4 : Constant  Value=7.50
  Divide : Product  Inputs=*/
  Math Function : Math  Operator=pow
  Product : Product
  Square : Math  Operator=square
  Subtract : Sum  Inputs=+-
  CI : Outport
  wires:
  C3/1 -> Subtract/2
  moisture[%]/1 -> Subtract/1
  Subtract/1 -> Square/1
  Square/1 -> Add/2
  C2/1 -> Add/1
  Add/1 -> Divide/2
  density[g/cm3]/1 -> Math Function/1
  C4/1 -> Math Function/2
  Math Function/1 -> Product/2
  C1/1 -> Product/1
  Product/1 -> Divide/1
  Divide/1 -> CI/1

== system Tractor_HIT_Discrete/WorkloadModel/Tires and Ground/CI_Calc/2 ==
  note: %CI=(C1*(DD^C4))/(C2+(MC-C3)^2) Ayers模型
  moisture[%] : Inport
  density[g/cm3] : Inport  Port=2
  Action Port : ActionPort  ActionPortLabel=elseif(u1 == 2)
  Add : Sum
  C1 : Constant  Value=1.10
  C2 : Constant  Value=2.19
  C3 : Constant  Value=3.29
  C4 : Constant  Value=9.34
  Divide : Product  Inputs=*/
  Math Function : Math  Operator=pow
  Product : Product
  Square : Math  Operator=square
  Subtract : Sum  Inputs=+-
  CI : Outport
  wires:
  C3/1 -> Subtract/2
  moisture[%]/1 -> Subtract/1
  Subtract/1 -> Square/1
  Square/1 -> Add/2
  C2/1 -> Add/1
  Add/1 -> Divide/2
  density[g/cm3]/1 -> Math Function/1
  C4/1 -> Math Function/2
  Math Function/1 -> Product/2
  C1/1 -> Product/1
  Product/1 -> Divide/1
  Divide/1 -> CI/1

== system Tractor_HIT_Discrete/WorkloadModel/Tires and Ground/CI_Calc/If Action Subsystem ==
  note: %CI=(C1*(DD^C4))/(C2+(MC-C3)^2) Ayers模型
  moisture[%] : Inport
  density[g/cm3] : Inport  Port=2
  Scene[-] : Inport  Port=3
  Action Port : ActionPort  ActionPortLabel=if(u1 == 0)
  Add : Sum
  C1 : Constant  Value=928.1
  C2 : Constant  Value=20.22
  C3 : Constant  Value=47.41
  C4 : Constant  Value=6.60
  C5 : Constant  Value=7.41
  Divide : Product  Inputs=*/
  Math Function : Math  Operator=pow
  Product : Product
  Square : Math  Operator=square
  Subtract : Sum  Inputs=+-
  Switch : Switch  Criteria=u2 > Threshold  SaturateOnIntegerOverflow=off  InputSameDT=off
  CI : Outport
  wires:
  moisture[%]/1 -> Subtract/1
  Subtract/1 -> Square/1
  Square/1 -> Add/2
  C2/1 -> Add/1
  Add/1 -> Divide/2
  density[g/cm3]/1 -> Math Function/1
  C4/1 -> Math Function/2
  Math Function/1 -> Product/2
  C1/1 -> Product/1
  Product/1 -> Divide/1
  Divide/1 -> CI/1
  Scene[-]/1 -> Switch/2
  C3/1 -> Switch/3  "paddy"
  C5/1 -> Switch/1  "dry"
  Switch/1 -> Subtract/2

== system Tractor_HIT_Discrete/WorkloadModel/Tires and Ground/CI_Calc/If Action Subsystem1 ==
  note: %CI=(C1*(DD^C4))/(C2+(MC-C3)^2) Ayers模型
  moisture[%] : Inport
  density[g/cm3] : Inport  Port=2
  Action Port : ActionPort  ActionPortLabel=elseif(u1 == 1)
  Add : Sum
  C1 : Constant  Value=928.1
  C2 : Constant  Value=20.22
  C3 : Constant  Value=6.41
  C4 : Constant  Value=6.60
  Divide : Product  Inputs=*/
  Math Function : Math  Operator=pow
  Product : Product
  Square : Math  Operator=square
  Subtract : Sum  Inputs=+-
  CI : Outport
  wires:
  Divide/1 -> CI/1
  Product/1 -> Divide/1
  C1/1 -> Product/1
  Math Function/1 -> Product/2
  C4/1 -> Math Function/2
  density[g/cm3]/1 -> Math Function/1
  Add/1 -> Divide/2
  C2/1 -> Add/1
  Square/1 -> Add/2
  Subtract/1 -> Square/1
  moisture[%]/1 -> Subtract/1
  C3/1 -> Subtract/2

== system Tractor_HIT_Discrete/WorkloadModel/Tires and Ground/F_longitudinal_Calc_single/PaddyLand ==
  Fz_f[N] : Inport
  Fz_r[N] : Inport  Port=2
  S_f : Inport  Port=3
  S_r : Inport  Port=4
  Constant : Constant
  Constant1 : Constant
  Gain : Gain  Gain=0.01
  Gain1 : Gain  Gain=0.02
  Product{,1..3} (4 alike) : Product  Inputs=3
  Subtract : Sum  Inputs=+-
  Subtract1 : Sum  Inputs=+-
  miu : Constant  Value=0.8
  ro : Constant  Value=0.1
  FR_f[N] : Outport
  FR_r[N] : Outport  Port=2
  FX_f[N] : Outport  Port=3
  FX_r[N] : Outport  Port=4
  wires:
  Product2/1 -> FR_f[N]/1
  Product3/1 -> FR_r[N]/1
  miu/1 -> Product1/1, Product/1
  Product/1 -> FX_f[N]/1
  Product1/1 -> FX_r[N]/1
  ro/1 -> Product2/1, Product3/1
  Fz_f[N]/1 -> Product2/2, Product/2
  Fz_r[N]/1 -> Product3/2, Product1/2
  S_r/1 -> Gain1/1
  S_f/1 -> Gain/1
  Constant/1 -> Subtract/1
  Gain1/1 -> Subtract/2
  Gain/1 -> Subtract1/2
  Constant1/1 -> Subtract1/1
  Subtract1/1 -> Product/3, Product2/3
  Subtract/1 -> Product1/3, Product3/3

== system Tractor_HIT_Discrete/WorkloadModel/Tires and Ground/F_longitudinal_Calc_single/WheelSpdCalc ==
  DriveCmd [-] : Inport
  VehSpd[m/s] : Inport  Port=2
  T_Wf [Nm] : Inport  Port=3
  T_Wr [Nm] : Inport  Port=4
  Fx_f[N] : Inport  Port=5
  Fx_r[N] : Inport  Port=6
  Discrete-Time Integrator : DiscreteIntegrator  SampleTime=-1  LimitOutput=on  UpperSaturationLimit=3  LowerSaturationLimit=0  ICPrevOutput=DiscIntNeverNeededParam  ICPrevScaledInput=DiscIntNeverNeededParam
  Discrete-Time Integrator1 : DiscreteIntegrator  SampleTime=-1  LimitOutput=on  UpperSaturationLimit=3  LowerSaturationLimit=0  ICPrevOutput=DiscIntNeverNeededParam  ICPrevScaledInput=DiscIntNeverNeededParam
  Gain : Gain  Gain=Rf
  Gain1 : Gain  Gain=Rr
  Gain2 : Gain  Gain=1/Jr
  Gain3 : Gain  Gain=1/Jf
  Gain7 : Gain  Gain=Rf
  Gain8 : Gain  Gain=Rr
  Saturation : Saturate  UpperLimit=2  LowerLimit=-1
  Saturation1 : Saturate  UpperLimit=2  LowerLimit=-1
  Subtract2 : Sum  Inputs=+-
  Subtract4 : Sum  Inputs=+-
  Switch : Switch  Criteria=u2 ~= 0  SaturateOnIntegerOverflow=off  InputSameDT=off
  WhlSpdF[m/s] : Outport
  WhlSpdR[m/s] : Outport  Port=2
  wires:
  Fx_r[N]/1 -> Gain1/1
  Saturation1/1 -> Discrete-Time Integrator/1
  Discrete-Time Integrator/1 -> Gain7/1
  Saturation/1 -> Discrete-Time Integrator1/1
  Switch/1 -> WhlSpdF[m/s]/1
  Gain8/1 -> WhlSpdR[m/s]/1
  Gain7/1 -> Switch/1  "4WD"
  DriveCmd [-]/1 -> Switch/2
  Discrete-Time Integrator1/1 -> Gain8/1
  T_Wf [Nm]/1 -> Subtract4/1
  Fx_f[N]/1 -> Gain/1
  Gain3/1 -> Saturation1/1
  VehSpd[m/s]/1 -> Switch/3  "RWD"
  Gain2/1 -> Saturation/1
  Gain/1 -> Subtract4/2
  Gain1/1 -> Subtract2/2
  T_Wr [Nm]/1 -> Subtract2/1
  Subtract4/1 -> Gain3/1
  Subtract2/1 -> Gain2/1

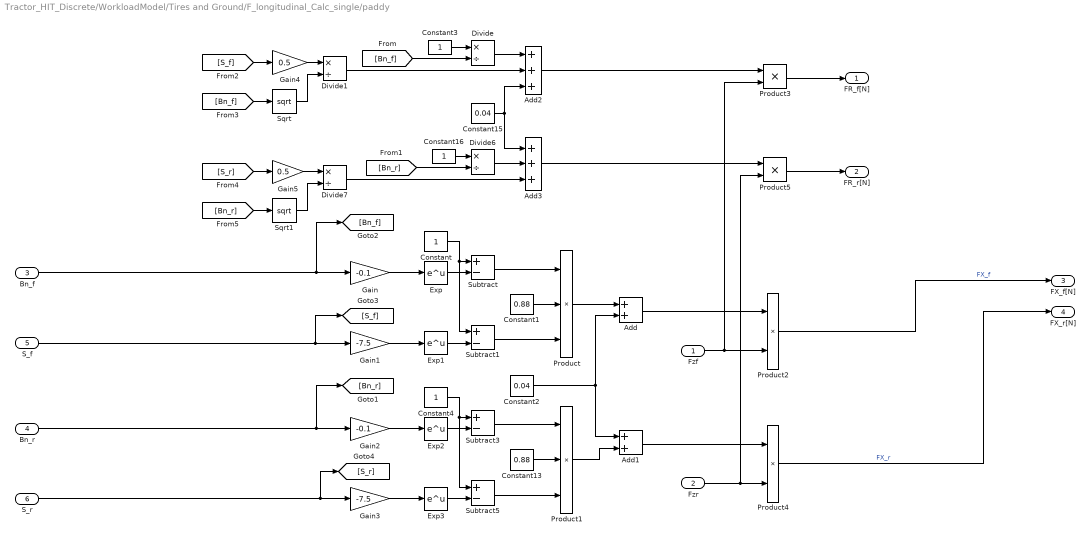
== system Tractor_HIT_Discrete/WorkloadModel/Tires and Ground/F_longitudinal_Calc_single/paddy ==
  Fzf : Inport
  Fzr : Inport  Port=2
  Bn_f : Inport  Port=3
  Bn_r : Inport  Port=4
  S_f : Inport  Port=5
  S_r : Inport  Port=6
  Add : Sum
  Add1 : Sum
  Add2 : Sum  Inputs=+++
  Add3 : Sum  Inputs=+++
  Constant{,3..4,16} (4 alike) : Constant
  Constant1 : Constant  Value=0.88
  Constant13 : Constant  Value=0.88
  Constant15 : Constant  Value=0.04
  Constant2 : Constant  Value=0.04
  Divide{,1,6..7} (4 alike) : Product  Inputs=*/
  Exp{,1..3} (4 alike) : Math
  Gain : Gain  Gain=-0.1
  Gain1 : Gain  Gain=-7.5
  Gain2 : Gain  Gain=-0.1
  Gain3 : Gain  Gain=-7.5
  Gain4 : Gain  Gain=0.5
  Gain5 : Gain  Gain=0.5
  Product : Product  Inputs=3
  Product1 : Product  Inputs=3
  Product{2..5} (4 alike) : Product
  Sqrt : Sqrt
  Sqrt1 : Sqrt
  Subtract{,1,3,5} (4 alike) : Sum  Inputs=+-
  FR_f[N] : Outport
  FR_r[N] : Outport  Port=2
  FX_f[N] : Outport  Port=3
  FX_r[N] : Outport  Port=4
  wires:
  Product4/1 -> FX_r[N]/1  "FX_r"
  Exp3/1 -> Subtract5/2
  Divide1/1 -> Add2/2
  Product2/1 -> FX_f[N]/1  "FX_f"
  Constant16/1 -> Divide6/1
  Divide7/1 -> Add3/3
  [S_r] -> Gain5/1
  Sqrt1/1 -> Divide7/2
  Product/1 -> Add/1
  [S_f] -> Gain4/1
  [Bn_r] -> Divide6/2
  Gain4/1 -> Divide1/1
  Add2/1 -> Product3/1
  [Bn_f] -> Divide/2
  Add1/1 -> Product4/1
  Subtract5/1 -> Product1/3
  Bn_f/1 -> Gain/1, [Bn_f]
  Constant15/1 -> Add3/1, Add2/3
  [Bn_r] -> Sqrt1/1
  S_r/1 -> Gain3/1, [S_r]
  Product1/1 -> Add1/2
  Fzr/1 -> Product4/2, Product5/2
  Exp2/1 -> Subtract3/2
  Gain/1 -> Exp/1
  Subtract3/1 -> Product1/1
  Constant2/1 -> Add/2, Add1/1
  Constant13/1 -> Product1/2
  Subtract/1 -> Product/1
  [Bn_f] -> Sqrt/1
  Constant4/1 -> Subtract3/1, Subtract5/1
  S_f/1 -> Gain1/1, [S_f]
  Gain2/1 -> Exp2/1
  Gain5/1 -> Divide7/1
  Constant3/1 -> Divide/1
  Product3/1 -> FR_f[N]/1
  Product5/1 -> FR_r[N]/1
  Constant/1 -> Subtract/1, Subtract1/1
  Gain3/1 -> Exp3/1
  Add/1 -> Product2/1
  Sqrt/1 -> Divide1/2
  Exp/1 -> Subtract/2
  Divide/1 -> Add2/1
  Divide6/1 -> Add3/2
  Constant1/1 -> Product/2
  Add3/1 -> Product5/1
  Gain1/1 -> Exp1/1
  Fzf/1 -> Product2/2, Product3/2
  Exp1/1 -> Subtract1/2
  Bn_r/1 -> Gain2/1, [Bn_r]
  Subtract1/1 -> Product/3
